simulink model "b0_foc_m"  (R2023b)
settings: Solver=FixedStepDiscrete  StartTime=0.0  StopTime=130  FixedStep=0.001  RelTol=1e-3
undefined symbols (not defined in the file or in its folder): DiscIntNeverNeededParam
settings Model: Creator=28447  LastModifiedBy=28447

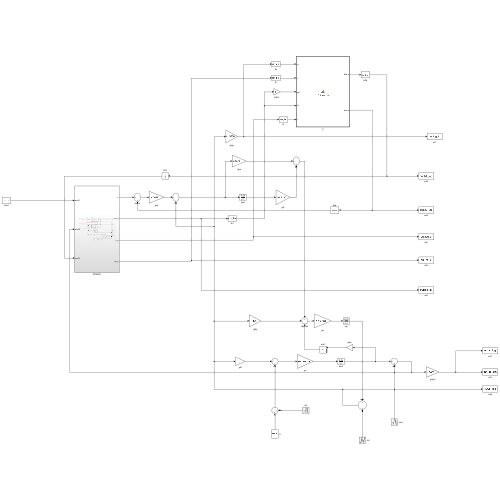
[thumbnail: Simulink's stored preview of the top-level diagram]
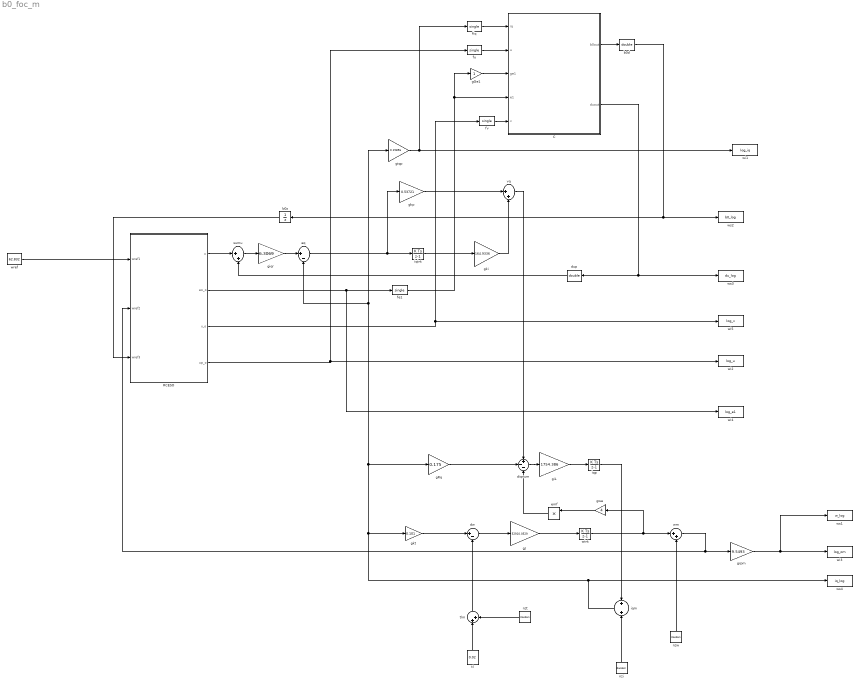
== system b0_foc_m ==
  C : MATLAB Function  TreatAsAtomicUnit=on
  RCESO : Subsystem
  b0d : DataTypeConversion  OutDataTypeStr=double  SaturateOnIntegerOverflow=off  RndMeth=Floor
  b0z : UnitDelay  InitialCondition=400  SampleTime=0.001  HasFrameUpgradeWarning=on
  diqnum : Sum  Inputs=+--
  dup : DataTypeConversion  OutDataTypeStr=double  SaturateOnIntegerOverflow=off  RndMeth=Floor
  dw : Sum  Inputs=|+-
  emf : Product  Inputs=3
  eq : Sum  Inputs=|+-
  fe1 : DataTypeConversion  OutDataTypeStr=single  SaturateOnIntegerOverflow=off  RndMeth=Floor
  fiq : DataTypeConversion  OutDataTypeStr=single  SaturateOnIntegerOverflow=off  RndMeth=Floor
  fu : DataTypeConversion  OutDataTypeStr=single  SaturateOnIntegerOverflow=off  RndMeth=Floor
  fv : DataTypeConversion  OutDataTypeStr=single  SaturateOnIntegerOverflow=off  RndMeth=Floor
  gGe1 : Gain
  gJ : Gain  Gain=52910.0529
  gRq : Gain  Gain=0.175
  giL : Gain  Gain=1754.386
  giqp : Gain  Gain=0.15856
  giqr : Gain  Gain=6.3069
  gki : Gain  Gain=164.9336
  gkp : Gain  Gain=0.53721
  gkt : Gain  Gain=0.101
  grpm : Gain  Gain=9.5493
  gwe : Gain  Gain=4
  iqint : DiscreteIntegrator  SampleTime=0.001  ICPrevOutput=DiscIntNeverNeededParam  ICPrevScaledInput=DiscIntNeverNeededParam
  iqm : Sum
  iqp : DiscreteIntegrator  SampleTime=0.001  ICPrevOutput=DiscIntNeverNeededParam  ICPrevScaledInput=DiscIntNeverNeededParam
  nzi : UniformRandomNumber  Minimum=-0.1  Maximum=0.1  Seed=23456  SampleTime=1e-3
  nzt : RandomNumber  Variance=0.0001  Seed=34567  SampleTime=1e-3
  nzw : RandomNumber  Variance=0.098696  Seed=12345  SampleTime=1e-3
  sumu : Sum  Inputs=|++
  tl : Constant  Value=0.02  SampleTime=0.001
  tlm : Sum  Inputs=|++
  vq : Sum  Inputs=|++
  wi1 : ToWorkspace  VariableName=log_iq  SaveFormat=Timeseries  SampleTime=0.001
  wi2 : ToWorkspace  VariableName=log_u  SaveFormat=Timeseries  SampleTime=0.001
  wi3 : ToWorkspace  VariableName=log_om  SaveFormat=Timeseries  SampleTime=0.001
  wi4 : ToWorkspace  VariableName=log_e1  SaveFormat=Timeseries  SampleTime=0.001
  wi5 : ToWorkspace  VariableName=log_v  SaveFormat=Timeseries  SampleTime=0.001
  wint : DiscreteIntegrator  SampleTime=0.001  ICPrevOutput=DiscIntNeverNeededParam  ICPrevScaledInput=DiscIntNeverNeededParam
  wm : Sum  Inputs=|++
  wref : Constant  Value=62.832  SampleTime=0.001
  ws1 : ToWorkspace  VariableName=w_log  SaveFormat=Timeseries  SampleTime=0.001
  ws2 : ToWorkspace  VariableName=b0_log  SaveFormat=Timeseries  SampleTime=0.001
  ws3 : ToWorkspace  VariableName=du_log  SaveFormat=Timeseries  SampleTime=0.001
  ws4 : ToWorkspace  VariableName=iq_log  SaveFormat=Timeseries  SampleTime=0.001
  wires:
  giqp/1 -> wi1/1, fiq/1
  RCESO/4(up_o) -> fu/1, wi2/1
  RCESO/2(eo_o) -> fe1/1, wi4/1
  RCESO/3(v_o) -> fv/1, wi5/1
  fiq/1 -> C/1(iq)
  fu/1 -> C/2(u)
  fe1/1 -> gGe1/1, C/4(e1)
  gGe1/1 -> C/3(ge1)
  fv/1 -> C/5(v)
  C/1(b0out) -> b0d/1
  b0d/1 -> ws2/1, b0z/1
  C/2(duout) -> ws3/1, dup/1
  RCESO/1(u) -> sumu/1
  dup/1 -> sumu/2
  wref/1 -> RCESO/1(wref1)
  wm/1 -> grpm/1, RCESO/2(wref2)
  b0z/1 -> RCESO/3(wref3)
  sumu/1 -> giqr/1
  giqr/1 -> eq/1
  iqm/1 -> gkt/1, gRq/1, giqp/1, eq/2, ws4/1
  eq/1 -> iqint/1, gkp/1
  iqint/1 -> gki/1
  gkp/1 -> vq/1
  gki/1 -> vq/2
  vq/1 -> diqnum/1
  gRq/1 -> diqnum/2
  emf/1 -> diqnum/3
  diqnum/1 -> giL/1
  giL/1 -> iqp/1
  wint/1 -> wm/1, gwe/1
  gwe/1 -> emf/1
  gkt/1 -> dw/1
  tlm/1 -> dw/2
  dw/1 -> gJ/1
  gJ/1 -> wint/1
  nzw/1 -> wm/2
  iqp/1 -> iqm/1
  nzi/1 -> iqm/2
  tl/1 -> tlm/1
  nzt/1 -> tlm/2
  grpm/1 -> ws1/1, wi3/1

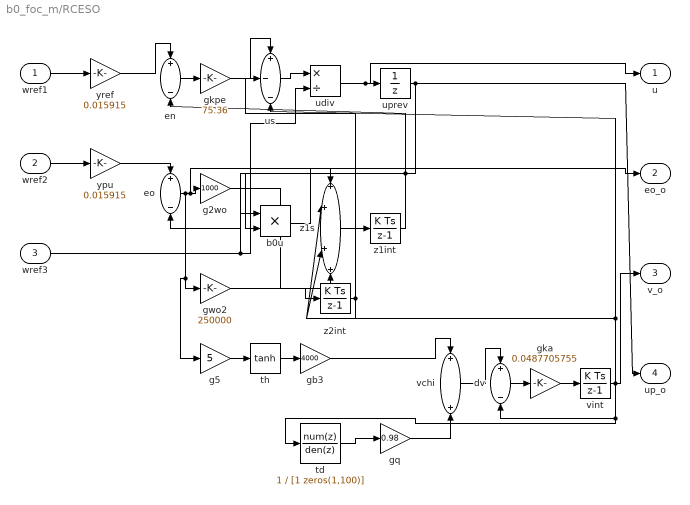
== system b0_foc_m/RCESO ==
  wref1 : Inport
  wref2 : Inport  Port=2
  wref3 : Inport  Port=3
  b0u : Product
  dv : Sum  Inputs=+-
  en : Sum  Inputs=+-
  eo : Sum  Inputs=+-
  g2wo : Gain  Gain=1000
  g5 : Gain  Gain=5
  gb3 : Gain  Gain=4000
  gka : Gain  Gain=0.0487705755
  gkpe : Gain  Gain=75.36
  gq : Gain  Gain=0.98
  gwo2 : Gain  Gain=250000
  td : DiscreteTransferFcn  Numerator=1  Denominator=[1 zeros(1,100)]  SampleTime=0.001
  th : Trigonometry  Operator=tanh
  udiv : Product  Inputs=*/
  uprev : UnitDelay  SampleTime=0.001  HasFrameUpgradeWarning=on
  us : Sum  Inputs=+--
  vchi : Sum
  vint : DiscreteIntegrator  SampleTime=0.001  ICPrevOutput=DiscIntNeverNeededParam  ICPrevScaledInput=DiscIntNeverNeededParam
  ypu : Gain  Gain=0.015915
  yref : Gain  Gain=0.015915
  z1int : DiscreteIntegrator  SampleTime=0.001  ICPrevOutput=DiscIntNeverNeededParam  ICPrevScaledInput=DiscIntNeverNeededParam
  z1s : Sum  Inputs=++++
  z2int : DiscreteIntegrator  SampleTime=0.001  ICPrevOutput=DiscIntNeverNeededParam  ICPrevScaledInput=DiscIntNeverNeededParam
  u : Outport
  eo_o : Outport  Port=2
  v_o : Outport  Port=3
  up_o : Outport  Port=4
  wires:
  ? -> ?
  wref1/1 -> yref/1
  wref2/1 -> ypu/1
  yref/1 -> en/1
  z1int/1 -> en/2, eo/2
  en/1 -> gkpe/1
  gkpe/1 -> us/1
  z2int/1 -> us/2, z1s/3
  vint/1 -> td/1, dv/2, us/3, z1s/2, v_o/1
  us/1 -> udiv/1
  wref3/1 -> udiv/2, b0u/1
  udiv/1 -> u/1, uprev/1
  uprev/1 -> up_o/1, b0u/2
  ypu/1 -> eo/1
  eo/1 -> gwo2/1, g5/1, eo_o/1, g2wo/1
  g2wo/1 -> z1s/4
  b0u/1 -> z1s/1
  z1s/1 -> z1int/1
  gwo2/1 -> z2int/1
  g5/1 -> th/1
  th/1 -> gb3/1
  td/1 -> gq/1
  gb3/1 -> vchi/1
  gq/1 -> vchi/2
  vchi/1 -> dv/1
  dv/1 -> gka/1
  gka/1 -> vint/1

== matlab function b0_foc_m/C ==
  data: iq input; u input; b0out output; ge1 input; e1 input; v input; duout output
function [b0out, duout] = b0_ident_m(iq, u, ge1, e1, v)
%#codegen
% 两段式高频注入 b0 在线辨识 —— MATLAB 版（配合 MATLAB Function 块，无需 C 编译器）
% 与 b0_ident.c 逐行等价：R2018b 及以后版本均可用
% ==================== 顶层可调参数（移植时只改这里）====================
dT     = 1e-3;      % 采样周期 [s]
f_inj  = 65;        % 注入频率 [Hz]：须为 5 Hz 整数倍，且约等于 6.5 x 机械频率
amp    = 0.118;     % 注入幅值 [pu]，上限 0.25
wave   = 0;         % 注入波形：0=正弦 1=方波 2=三角（三者峰值均为 1）
b0_init= 400;       % b0 初值，填控制器的标称值
b0lo   = 200;       % 硬下限（防发散）
b0hi   = 800;       % 硬上限
wo     = 500;       % 观测器带宽 [rad/s]，必须与 ESO 一致
kp     = 75.36;     % 转速环比例增益
% ---- 反演用的增益由外部输入 ge1 提供（G(e1) 在块外计算）----
% 第 3 个入参 ge1 即 G(e1)：线性 ESO 时 ge1 = e1；类 fal 时由外部 G 块给出。
% ---- 识别使能：0 = 只注入不更新 b0（关闭识别，用于对照）----
upd_on  = 1;
% ---- 运行使能：转速门限已移除（omega 不再作为入参，门限请在块外用使能信号实现）----
% ==================== 派生量（不要手改）====================
cyc    = f_inj*dT;          % 每拍相位增量 [周期]
wh     = 2*pi*f_inj;        % 注入角频率 [rad/s]
nseg   = round(0.2/dT);     % 段长 0.2 s 对应的拍数
% ---- 辨识调度 ----
warm   = 3;         % 预热 burst 数：前几次估计直接采用
nident = 24;        % 辨识 burst 总数：24 x 5 s = 120 s
nfrz   = 12;        % 冻结时取最近 12 次（60 s）均值：末 12 个覆盖 60–120 s
% ---- 门控：平台 + 陡降 + 软底 ----
d1     = 0.10;      % 平台半宽（偏离 <=10% 不衰减）
d2     = 0.20;      % 陡降宽度
dmax   = 0.50;      % 软底拐点（超过后权重不再下降）
abase  = 0.30;      % 基增益 alpha
mu     = 0.35;      % 基线滑动速率
% 一致性检查：cyc*nseg 必须是整数，否则段内不相干。
% 注意：MATLAB Function 块里不能放顶层 error() 断言——会让块的输出维度推断失败
% （"无法沿循环求取信号维度"），此检查只保留在 C 版与移植文档里。
cyc_nseg = cyc*nseg;   % 移植时人工确认该值为整数（65 Hz x 0.2 s = 13）
persistent init ph acc nacc seg active tick nxtick tstart d0 u0 q0 t0
persistent b0v goal gv base bvalid nest blast nblast nburst frozen
persistent pdC sdC lpa b1 b2 bc
if isempty(init)
    init = 1; ph = 0;
    acc = zeros(1,14); nacc = 0; seg = 0; active = 0;   % 11-14: SDFT(G1(e1)), SDFT(G2(e1))
    tick = 0; nxtick = 1; tstart = 0;      % 整数拍时基（与 C 版一致）
    d0 = 0; u0 = 0; q0 = 0; t0 = 1;
    b0v = b0_init; goal = b0_init; gv = 0;
    base = 0; bvalid = 0; nest = 0;
    blast = zeros(1,12); nblast = 0; nburst = 0; frozen = 0;
    % ---- 派生常量（只算一次）----
    b1 = 2*wo;                       % beta1 = 2*wo*kappa1，delta=1 时 kappa1=1
    b2 = wo*wo;                      % beta2 = wo^2*kappa2，delta=1 时 kappa2=1
    sdC = (exp(1i*wh*dT) - 1) / dT;
    pdC = sdC + b1 + b2/sdC;
    bc  = b2/sdC;                    % beta2/Sd（精确反演用，只算一次）
    tau = 50/kp;                     % b0 低通时间常数 = 50/kp = 0.663 s（与 C 版一致）
    lpa = 1 - exp(-dT/tau);          % 低通系数，每拍执行一次
end
% （参数已移至函数开头，见上方“顶层可调参数”）
% ---- 相位推进 ----
ph = ph + cyc;
if ph >= 1, ph = ph - 1; end
c = cos(2*pi*ph); s = sin(2*pi*ph);
% ---- b0 低通（每拍） ----
if gv ~= 0
    b0v = b0v + lpa*(goal - b0v);
    if abs(goal - b0v) <= 1e-4*abs(goal)
        b0v = goal; gv = 0;
    end
end
% ---- 调度 ----
tick = tick + 1;                        % 整数拍计数：不漂
du = 0;
if (~active) && (~frozen) && (tick >= nxtick)
    active = 1; seg = 0; nacc = 0; acc(:) = 0;
    tstart = tick;                      % 周期按 burst 起点计
end
if active
    acc(1) = acc(1) + e1*c;  acc(2) = acc(2) + e1*s;
    acc(3) = acc(3) + v*c;   acc(4) = acc(4) + v*s;
    acc(5) = acc(5) + u*c;   acc(6) = acc(6) + u*s;
    acc(7) = acc(7) + iq*c;  acc(8) = acc(8) + iq*s;
    % G(e1) 由外部输入 ge1 提供（不在块内推导）
    acc(11)= acc(11)+ ge1*c;  acc(12)= acc(12)+ ge1*s;
    acc(13)= acc(13)+ ge1*c;  acc(14)= acc(14)+ ge1*s;
    if seg == 1
        % 波形（峰值=1，与 C 版 b0_wave_value 一致）
        if wave == 1
            if s >= 0, wv = 1; else, wv = -1; end
        elseif wave == 2
            a4 = ph*4;
            if a4 < 1,        wv = a4;
            elseif a4 < 3,    wv = 2 - a4;
            else,             wv = a4 - 4;
            end
        else
            wv = s;
        end
        du = amp*wv;
    end
    nacc = nacc + 1;
    if nacc >= nseg
        k = 2/nacc;
        E1 = k*(acc(1) - 1i*acc(2));
        Vc = k*(acc(3) - 1i*acc(4));
        Uc = k*(acc(5) - 1i*acc(6));
        Qc = k*(acc(7) - 1i*acc(8));
        % 代数恒等式（只依赖观测器方程，不含任何线性化）：
        %   d^ = V + Sd*E1 + beta1*SDFT(G1(e1)) + (beta2/Sd)*SDFT(G2(e1))
        % 线性观测器时 G1=G2=e1，自动退化为 V + (Sd+beta1+beta2/Sd)*E1
        G1c = k*(acc(11) - 1i*acc(12));
        G2c = k*(acc(13) - 1i*acc(14));
        D  = Vc + sdC*E1 + b1*G1c + bc*G2c;
        if abs(Uc) > 1e-9, T = Qc/Uc; else, T = 1; end
        if seg == 0
            d0 = D; u0 = Uc; q0 = Qc; t0 = T;
            seg = 1;
        else
            num = (D - d0) + b0v*(Uc - u0);
            den = Qc - q0;
            if abs(den) > 1e-9
                bq = abs(num/den);              % 取模长：对相位误差免疫
                bq = min(max(bq, b0lo), b0hi);
                if upd_on == 0
                    % 识别关闭：只算 bq，不更新 b0（b0 停在 b0_init）
                elseif ~bvalid
                    base = bq; bvalid = 1; goal = bq; gv = 1; nest = 1;   % 经低通
                elseif nest < warm
                    base = bq; goal = bq; gv = 1; nest = nest + 1;        % 经低通
                else
                    dd = abs(bq - base)/max(abs(base),1e-9);
                    if dd <= d1
                        w = 1;
                    elseif dd <= dmax
                        w = exp(-(dd - d1)/max(d2,1e-9));
                    else
                        w = exp(-(dmax - d1)/max(d2,1e-9));
                    end
                    goal = b0v + abase*w*(bq - b0v); gv = 1;
                    base = base + mu*(bq - base);
                    nest = nest + 1;
                end
                if upd_on == 0
                    % 识别关闭：不记录、不冻结
                elseif nblast < nfrz
                    nblast = nblast + 1; blast(nblast) = bq;
                else
                    blast(1:nfrz-1) = blast(2:nfrz); blast(nfrz) = bq;
                end
            end
            active = 0;
            nburst = nburst + 1;
            if (upd_on ~= 0) && (nburst >= nident)
                b0v = mean(blast(1:max(nblast,1)));
                goal = b0v; gv = 0; frozen = 1; nxtick = tick + round(3600/dT);
            else
                nxtick = tstart + round(5/dT);        % 5 s 起点周期
            end
            seg = 0;
        end
        acc(:) = 0; nacc = 0;
    end
end
b0out = b0v;
duout = du;
end
